simulink model "beaver_agent_env_ground_autobrake_steering"  (R2022a)
settings: Solver=ode15s  StartTime=0.0  StopTime=30  FixedStep=1/120  MaxStep=0.005  RelTol=1e-6  AbsTol=1e-8
PreLoadFcn:
  | [aircraft, state] = astDehavillandBeaver();
  | thrustX = getCoefficient(aircraft,"CX","Propeller",Component="Propeller");
  | AileronCmd = 0.00202547955338193;
  | ElevatorCmd = -0.0109658218633661;
  | RudderCmd = -0.0374364069557001;
  | Throttle_Left = 0.16863024396043;
  | Throttle_Right = 0.16863024396043;
  | NoseWheelSteerCmdData = timeseries(0,0);
  | GearDownCmd = 1; RunwayMu = 0.65;
  | GroundMass = state.Mass;
  | GroundCrr = 0.015; GroundSideVGain = 0.35;
  | GroundYawGain = 0.15; GroundSteerGain = 0.8; NoseGearArm = 2.4;
  | 
  | Throttle_Left=0; Throttle_Right=0;
  | AileronCmd=0; ElevatorCmd=0; RudderCmd=0;
  | NoseWheelSteerCmdData=timeseries([0;0],[0;60]);
model workspace (MATLAB code in the model file + MAT data in the model file):
  GroundStatic : object (value not decoded)
  inputs0 : object (value not decoded)
  states : object (value not decoded)
  states0 : object (value not decoded)
  other statements: initialize6DOFSkyHogg;
symbols that are objects in the model workspace (value not decoded): GroundStatic
undefined symbols (not defined in the file): aircraft, Earth, F, Light, MIL, state, WGS84
libraries: simulink x5, shared6dof x1, aerolibadyn x1, aerolibasang x1, aerolibatmos2 x1, aerolibwind2 x1, aerolibtransform2 x1, sharedtransform x1
(part 3 of 3)

== system beaver_agent_env_ground_autobrake_steering/GroundContactTireSteering/ThreePointGroundDynamics/RightMainGear/NormalReaction ==
  CompressionRate : Inport
  ContactGate : Inport  Port=2
  PositiveCompression : Inport  Port=3
  GearDown : Inport  Port=4
  ActiveContact : Product  Inputs=**
  DamperLoad : Gain  Gain=GroundStatic.NormalDamping(3)
  NoTensileNormalForce : Saturate  UpperLimit=inf  LowerLimit=0
  NormalForce : Product  Inputs=***
  SpringDamperLoad : Sum
  SpringLoad : Gain  Gain=GroundStatic.NormalStiffness(3)
  NormalForce_1 : Outport
  ActiveContact_1 : Outport  Port=2
  wires:
  ActiveContact/1 -> ActiveContact_1/1
  DamperLoad/1 -> SpringDamperLoad/2
  PositiveCompression/1 -> SpringLoad/1
  SpringDamperLoad/1 -> NoTensileNormalForce/1
  NormalForce/1 -> NormalForce_1/1
  CompressionRate/1 -> DamperLoad/1
  SpringLoad/1 -> SpringDamperLoad/1
  NoTensileNormalForce/1 -> NormalForce/1
  ContactGate/1 -> ActiveContact/1, NormalForce/2
  GearDown/1 -> ActiveContact/2, NormalForce/3

== system beaver_agent_env_ground_autobrake_steering/GroundContactTireSteering/ThreePointGroundDynamics/RightMainGear/TireFrictionCircle ==
  BrakeCommand : Inport
  WheelLongVelocity : Inport  Port=2
  WheelSideVelocity : Inport  Port=3
  NormalForce : Inport  Port=4
  RunwayMu : Inport  Port=5
  NormalForce_1 : Inport  Port=6
  BrakeCoefficient : Gain  Gain=GroundStatic.BrakeCoefficient
  CapacityRatio : Product  Inputs=*/
  FrictionCapacity : Product  Inputs=**
  FrictionCircleScale : Saturate  UpperLimit=1  LowerLimit=0
  LongCoefficient : Sum
  LongSlipSmooth : Trigonometry  Operator=tanh
  LongTireForce : Product  Inputs=**
  LongVelocityScale : Gain  Gain=1/GroundStatic.TireVelocityScale
  RawLong2 : Product  Inputs=**
  RawLongForce : Gain  Gain=-1
  RawLongForcePositive : Product  Inputs=***
  RawSide2 : Product  Inputs=**
  RawSideForce : Gain  Gain=-GroundStatic.TireLateralCoefficient
  RawSideForcePositive : Product  Inputs=**
  RollingCoefficient : Constant  Value=GroundStatic.RollingCoefficient
  SafeTireMagnitude : Saturate  UpperLimit=inf  LowerLimit=1e-8
  SideSlipSmooth : Trigonometry  Operator=tanh
  SideTireForce : Product  Inputs=**
  SideVelocityScale : Gain  Gain=1/GroundStatic.TireVelocityScale
  TireMagnitude : Sqrt
  TireMagnitude2 : Sum
  LongTireForce_1 : Outport
  SideTireForce_1 : Outport  Port=2
  wires:
  SideTireForce/1 -> SideTireForce_1/1
  RawLongForce/1 -> LongTireForce/1, RawLong2/1, RawLong2/2
  NormalForce_1/1 -> FrictionCapacity/2
  SafeTireMagnitude/1 -> CapacityRatio/2
  FrictionCircleScale/1 -> SideTireForce/2, LongTireForce/2
  RunwayMu/1 -> FrictionCapacity/1
  WheelLongVelocity/1 -> LongVelocityScale/1
  LongTireForce/1 -> LongTireForce_1/1
  LongVelocityScale/1 -> LongSlipSmooth/1
  FrictionCapacity/1 -> CapacityRatio/1
  TireMagnitude/1 -> SafeTireMagnitude/1
  BrakeCoefficient/1 -> LongCoefficient/2
  RawLongForcePositive/1 -> RawLongForce/1
  LongSlipSmooth/1 -> RawLongForcePositive/3
  WheelSideVelocity/1 -> SideVelocityScale/1
  LongCoefficient/1 -> RawLongForcePositive/2
  RawLong2/1 -> TireMagnitude2/1
  RawSideForcePositive/1 -> RawSideForce/1
  CapacityRatio/1 -> FrictionCircleScale/1
  SideSlipSmooth/1 -> RawSideForcePositive/2
  TireMagnitude2/1 -> TireMagnitude/1
  RawSide2/1 -> TireMagnitude2/2
  NormalForce/1 -> RawLongForcePositive/1, RawSideForcePositive/1
  RollingCoefficient/1 -> LongCoefficient/1
  SideVelocityScale/1 -> SideSlipSmooth/1
  BrakeCommand/1 -> BrakeCoefficient/1
  RawSideForce/1 -> SideTireForce/1, RawSide2/2, RawSide2/1

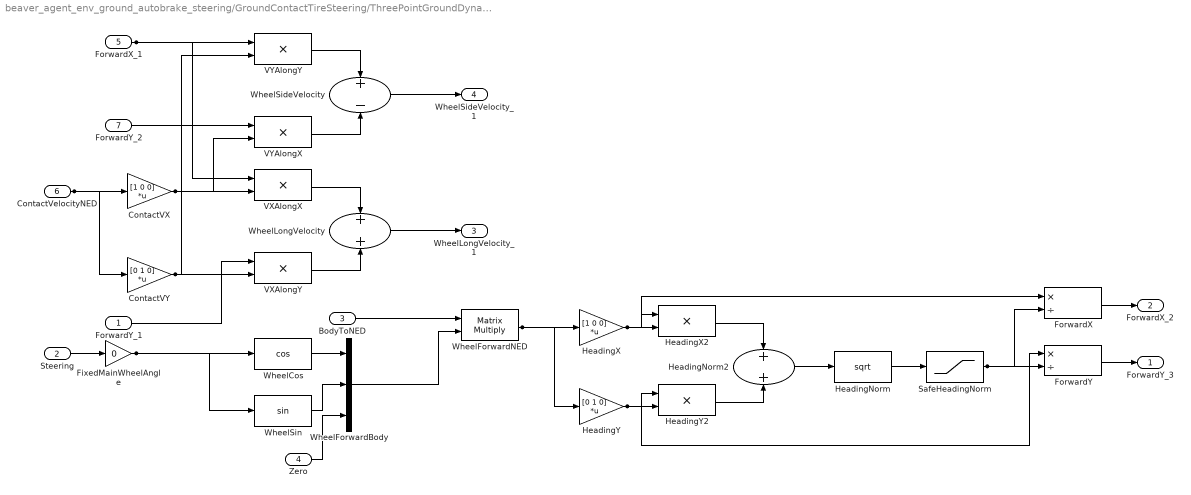
== system beaver_agent_env_ground_autobrake_steering/GroundContactTireSteering/ThreePointGroundDynamics/RightMainGear/WheelKinematics ==
  ForwardY_1 : Inport
  Steering : Inport  Port=2
  BodyToNED : Inport  Port=3
  Zero : Inport  Port=4
  ForwardX_1 : Inport  Port=5
  ContactVelocityNED : Inport  Port=6
  ForwardY_2 : Inport  Port=7
  ContactVX : Gain  Gain=[1 0 0]  Multiplication=Matrix(K*u)
  ContactVY : Gain  Gain=[0 1 0]  Multiplication=Matrix(K*u)
  FixedMainWheelAngle : Gain  Gain=0
  ForwardX : Product  Inputs=*/
  ForwardY : Product  Inputs=*/
  HeadingNorm : Sqrt
  HeadingNorm2 : Sum
  HeadingX : Gain  Gain=[1 0 0]  Multiplication=Matrix(K*u)
  HeadingX2 : Product  Inputs=**
  HeadingY : Gain  Gain=[0 1 0]  Multiplication=Matrix(K*u)
  HeadingY2 : Product  Inputs=**
  SafeHeadingNorm : Saturate  UpperLimit=inf  LowerLimit=1e-8
  VXAlongX : Product  Inputs=**
  VXAlongY : Product  Inputs=**
  VYAlongX : Product  Inputs=**
  VYAlongY : Product  Inputs=**
  WheelCos : Trigonometry  Operator=cos
  WheelForwardBody : Mux  Inputs=3
  WheelForwardNED : Product  Inputs=**  Multiplication=Matrix(*)
  WheelLongVelocity : Sum
  WheelSideVelocity : Sum  Inputs=+-
  WheelSin : Trigonometry
  ForwardY_3 : Outport
  ForwardX_2 : Outport  Port=2
  WheelLongVelocity_1 : Outport  Port=3
  WheelSideVelocity_1 : Outport  Port=4
  wires:
  BodyToNED/1 -> WheelForwardNED/1
  WheelLongVelocity/1 -> WheelLongVelocity_1/1
  SafeHeadingNorm/1 -> ForwardY/2, ForwardX/2
  ContactVY/1 -> VYAlongY/2, VXAlongY/2
  Zero/1 -> WheelForwardBody/3
  ContactVelocityNED/1 -> ContactVY/1, ContactVX/1
  WheelSideVelocity/1 -> WheelSideVelocity_1/1
  WheelSin/1 -> WheelForwardBody/2
  ForwardY/1 -> ForwardY_3/1
  VXAlongY/1 -> WheelLongVelocity/2
  ForwardX_1/1 -> VYAlongY/1, VXAlongX/1
  HeadingX2/1 -> HeadingNorm2/1
  WheelForwardBody/1 -> WheelForwardNED/2
  VYAlongY/1 -> WheelSideVelocity/1
  ForwardY_1/1 -> VXAlongY/1
  VXAlongX/1 -> WheelLongVelocity/1
  HeadingNorm2/1 -> HeadingNorm/1
  ForwardY_2/1 -> VYAlongX/1
  WheelCos/1 -> WheelForwardBody/1
  Steering/1 -> FixedMainWheelAngle/1
  HeadingY2/1 -> HeadingNorm2/2
  VYAlongX/1 -> WheelSideVelocity/2
  HeadingNorm/1 -> SafeHeadingNorm/1
  ForwardX/1 -> ForwardX_2/1
  FixedMainWheelAngle/1 -> WheelSin/1, WheelCos/1
  WheelForwardNED/1 -> HeadingY/1, HeadingX/1
  HeadingX/1 -> HeadingX2/2, HeadingX2/1, ForwardX/1
  HeadingY/1 -> HeadingY2/2, HeadingY2/1, ForwardY/1
  ContactVX/1 -> VYAlongX/2, VXAlongX/2

== system beaver_agent_env_ground_autobrake_steering/Aerodynamic Model/Aerodynamic Coefficients/Body Rate Damping/Subsystem/Divide ==
  Numerator : Inport
  TrueAirspeed : Inport  Port=2
  NonzeroAirspeed : Saturate  UpperLimit=inf  LowerLimit=GroundStatic.AirSpeedFloor
  OriginalDivision : Product  Inputs=*/
  NormalizedRate : Outport
  wires:
  TrueAirspeed/1 -> NonzeroAirspeed/1
  OriginalDivision/1 -> NormalizedRate/1
  NonzeroAirspeed/1 -> OriginalDivision/2
  Numerator/1 -> OriginalDivision/1

== system beaver_agent_env_ground_autobrake_steering/Aerodynamic Model/Aerodynamic Coefficients/Body Rate Damping/Subsystem/Product ==
  Numerator : Inport
  TrueAirspeed : Inport  Port=2
  NonzeroAirspeed : Saturate  UpperLimit=inf  LowerLimit=GroundStatic.AirSpeedFloor
  OriginalDivision : Product  Inputs=*/
  NormalizedRate : Outport
  wires:
  TrueAirspeed/1 -> NonzeroAirspeed/1
  OriginalDivision/1 -> NormalizedRate/1
  Numerator/1 -> OriginalDivision/1
  NonzeroAirspeed/1 -> OriginalDivision/2

== system beaver_agent_env_ground_autobrake_steering/GroundContactTireSteering/ThreePointGroundDynamics/LeftMainGear/ContactGeometry/ContactRotationVelocity ==
  A : Inport
  B : Inport  Port=2
  C1 : Sum  Inputs=+-
  C2 : Sum  Inputs=+-
  C3 : Sum  Inputs=+-
  DemuxA : Demux  Outputs=3
  DemuxB : Demux  Outputs=3
  N1 : Product  Inputs=**
  N2 : Product  Inputs=**
  N3 : Product  Inputs=**
  P1 : Product  Inputs=**
  P2 : Product  Inputs=**
  P3 : Product  Inputs=**
  Result : Mux  Inputs=3
  AxB : Outport
  wires:
  C1/1 -> Result/1
  Result/1 -> AxB/1
  P3/1 -> C3/1
  C3/1 -> Result/3
  C2/1 -> Result/2
  N3/1 -> C3/2
  N2/1 -> C2/2
  P2/1 -> C2/1
  N1/1 -> C1/2
  P1/1 -> C1/1
  B/1 -> DemuxB/1
  A/1 -> DemuxA/1
  DemuxA/1 -> N2/1, P3/1
  DemuxB/1 -> P2/2, N3/2
  DemuxB/3 -> P1/2, N2/2
  DemuxB/2 -> N1/2, P3/2
  DemuxA/2 -> P1/1, N3/1
  DemuxA/3 -> N1/1, P2/1

== system beaver_agent_env_ground_autobrake_steering/GroundContactTireSteering/ThreePointGroundDynamics/LeftMainGear/ContactGeometry/UncompressedPointRotationVelocity ==
  A : Inport
  B : Inport  Port=2
  C1 : Sum  Inputs=+-
  C2 : Sum  Inputs=+-
  C3 : Sum  Inputs=+-
  DemuxA : Demux  Outputs=3
  DemuxB : Demux  Outputs=3
  N1 : Product  Inputs=**
  N2 : Product  Inputs=**
  N3 : Product  Inputs=**
  P1 : Product  Inputs=**
  P2 : Product  Inputs=**
  P3 : Product  Inputs=**
  Result : Mux  Inputs=3
  AxB : Outport
  wires:
  P2/1 -> C2/1
  C1/1 -> Result/1
  Result/1 -> AxB/1
  DemuxA/2 -> P1/1, N3/1
  P3/1 -> C3/1
  N1/1 -> C1/2
  C3/1 -> Result/3
  DemuxA/1 -> N2/1, P3/1
  C2/1 -> Result/2
  N3/1 -> C3/2
  N2/1 -> C2/2
  P1/1 -> C1/1
  B/1 -> DemuxB/1
  A/1 -> DemuxA/1
  DemuxB/1 -> P2/2, N3/2
  DemuxB/3 -> P1/2, N2/2
  DemuxB/2 -> N1/2, P3/2
  DemuxA/3 -> N1/1, P2/1

== system beaver_agent_env_ground_autobrake_steering/GroundContactTireSteering/ThreePointGroundDynamics/NoseGear/ContactGeometry/ContactRotationVelocity ==
  A : Inport
  B : Inport  Port=2
  C1 : Sum  Inputs=+-
  C2 : Sum  Inputs=+-
  C3 : Sum  Inputs=+-
  DemuxA : Demux  Outputs=3
  DemuxB : Demux  Outputs=3
  N1 : Product  Inputs=**
  N2 : Product  Inputs=**
  N3 : Product  Inputs=**
  P1 : Product  Inputs=**
  P2 : Product  Inputs=**
  P3 : Product  Inputs=**
  Result : Mux  Inputs=3
  AxB : Outport
  wires:
  C1/1 -> Result/1
  Result/1 -> AxB/1
  P3/1 -> C3/1
  B/1 -> DemuxB/1
  C3/1 -> Result/3
  C2/1 -> Result/2
  N3/1 -> C3/2
  N2/1 -> C2/2
  P2/1 -> C2/1
  N1/1 -> C1/2
  P1/1 -> C1/1
  A/1 -> DemuxA/1
  DemuxA/2 -> P1/1, N3/1
  DemuxA/1 -> N2/1, P3/1
  DemuxB/2 -> N1/2, P3/2
  DemuxB/1 -> P2/2, N3/2
  DemuxA/3 -> N1/1, P2/1
  DemuxB/3 -> P1/2, N2/2

== system beaver_agent_env_ground_autobrake_steering/GroundContactTireSteering/ThreePointGroundDynamics/NoseGear/ContactGeometry/UncompressedPointRotationVelocity ==
  A : Inport
  B : Inport  Port=2
  C1 : Sum  Inputs=+-
  C2 : Sum  Inputs=+-
  C3 : Sum  Inputs=+-
  DemuxA : Demux  Outputs=3
  DemuxB : Demux  Outputs=3
  N1 : Product  Inputs=**
  N2 : Product  Inputs=**
  N3 : Product  Inputs=**
  P1 : Product  Inputs=**
  P2 : Product  Inputs=**
  P3 : Product  Inputs=**
  Result : Mux  Inputs=3
  AxB : Outport
  wires:
  C1/1 -> Result/1
  Result/1 -> AxB/1
  P3/1 -> C3/1
  C3/1 -> Result/3
  C2/1 -> Result/2
  N3/1 -> C3/2
  N2/1 -> C2/2
  P2/1 -> C2/1
  N1/1 -> C1/2
  P1/1 -> C1/1
  B/1 -> DemuxB/1
  A/1 -> DemuxA/1
  DemuxA/1 -> N2/1, P3/1
  DemuxB/1 -> P2/2, N3/2
  DemuxB/3 -> P1/2, N2/2
  DemuxB/2 -> N1/2, P3/2
  DemuxA/2 -> P1/1, N3/1
  DemuxA/3 -> N1/1, P2/1

== system beaver_agent_env_ground_autobrake_steering/GroundContactTireSteering/ThreePointGroundDynamics/RightMainGear/ContactGeometry/ContactRotationVelocity ==
  A : Inport
  B : Inport  Port=2
  C1 : Sum  Inputs=+-
  C2 : Sum  Inputs=+-
  C3 : Sum  Inputs=+-
  DemuxA : Demux  Outputs=3
  DemuxB : Demux  Outputs=3
  N1 : Product  Inputs=**
  N2 : Product  Inputs=**
  N3 : Product  Inputs=**
  P1 : Product  Inputs=**
  P2 : Product  Inputs=**
  P3 : Product  Inputs=**
  Result : Mux  Inputs=3
  AxB : Outport
  wires:
  C1/1 -> Result/1
  Result/1 -> AxB/1
  P3/1 -> C3/1
  C3/1 -> Result/3
  C2/1 -> Result/2
  N3/1 -> C3/2
  N2/1 -> C2/2
  P2/1 -> C2/1
  N1/1 -> C1/2
  P1/1 -> C1/1
  B/1 -> DemuxB/1
  A/1 -> DemuxA/1
  DemuxA/2 -> P1/1, N3/1
  DemuxA/1 -> N2/1, P3/1
  DemuxB/2 -> N1/2, P3/2
  DemuxB/1 -> P2/2, N3/2
  DemuxA/3 -> N1/1, P2/1
  DemuxB/3 -> P1/2, N2/2

== system beaver_agent_env_ground_autobrake_steering/GroundContactTireSteering/ThreePointGroundDynamics/RightMainGear/ContactGeometry/UncompressedPointRotationVelocity ==
  A : Inport
  B : Inport  Port=2
  C1 : Sum  Inputs=+-
  C2 : Sum  Inputs=+-
  C3 : Sum  Inputs=+-
  DemuxA : Demux  Outputs=3
  DemuxB : Demux  Outputs=3
  N1 : Product  Inputs=**
  N2 : Product  Inputs=**
  N3 : Product  Inputs=**
  P1 : Product  Inputs=**
  P2 : Product  Inputs=**
  P3 : Product  Inputs=**
  Result : Mux  Inputs=3
  AxB : Outport
  wires:
  Result/1 -> AxB/1
  P3/1 -> C3/1
  C3/1 -> Result/3
  C2/1 -> Result/2
  P2/1 -> C2/1
  DemuxB/1 -> P2/2, N3/2
  C1/1 -> Result/1
  N3/1 -> C3/2
  N2/1 -> C2/2
  DemuxA/3 -> N1/1, P2/1
  N1/1 -> C1/2
  P1/1 -> C1/1
  B/1 -> DemuxB/1
  A/1 -> DemuxA/1
  DemuxA/1 -> N2/1, P3/1
  DemuxB/2 -> N1/2, P3/2
  DemuxB/3 -> P1/2, N2/2
  DemuxA/2 -> P1/1, N3/1
